simulink library "lib_AC_MSG"  (R2026a)
settings: Solver=VariableStepAuto
undefined symbols (not defined in the file): block_buses, block_idx, buses_lf, fref, Lbiginv, MSGs_buses, Nbuses, op_MSG, Ps_lf
settings Model: Creator=atomas  LastModifiedBy=atomas

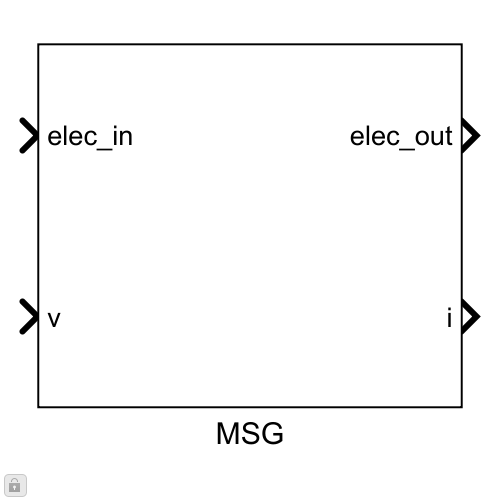
[thumbnail: Simulink's stored preview of the top-level diagram]
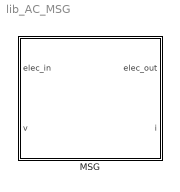
== system lib_AC_MSG ==
  MSG : Subsystem  mask(Doubly Fed Induction Generator){DFIGs_nodes=1, FBASE=50, D=0, H=7, Lssd_pu=1, Lssq_pu=0.6, Lmd_pu=0.9, Lmq_pu=0.5, Rs_pu=0.02, Lfd_pu=0.1, Rfd_pu=0.02, Rkd1_pu=10e6, Lkd1_pu=10e6, Rkd2_pu=10e6, Lkd2_pu=10e6, Rkq1_pu=10e6, Lkq1_pu=10e6, Rkq2_pu=10e6, Lkq2_pu=10e6, Rkq3_pu=10e6, Lkq3_pu=10e6, Ra_pu=0.008, La_pu=0.08, Cf_pu=0.0555, Ki_ia=0.1592, Kp_ia=9.1268e-04, Kid_m=1.9894, Kpd_m=0.0914, Kiq_m=1.1937, Kpq_m=0.0468, Ki_vc2=-0.1734, Kp_vc2=-0.0971, KPomegar=49, KIomegar=87.5, Kp_pll=9.1268e-05, Ki_pll=0.01592, T_e=1.15, T_1=12, T_2=1, T_A=0.01, K_A=200}
      mask prompts: FBASE "Base frequency (Hz)"; D "Damping (pu)"; H "Inertia (s)"; Lssd_pu "d-axis stator inductance (pu)"; Lssq_pu "q-axis stator inductance (pu)"; Lmd_pu "d-axis mutual inductance (pu)"; Lmq_pu "q-axis mutual inductance (pu)"; Rs_pu "Stator resistance (pu)"; Lfd_pu "Excitation indutance (pu)"; Rfd_pu "Excitation resistance (pu)"; Rkd1_pu "d-axis damper resistance 1 (pu)"; Lkd1_pu "d-axis damper inductance 1 (pu)"; Rkd2_pu "d-axis damper resistance 2 (pu)"; Lkd2_pu "d-axis damper inductance 2 (pu)"; Rkq1_pu "q-axis damper resistance 1(pu)"; Lkq1_pu "d-axis damper resistance 1 (pu)"; Rkq2_pu "d-axis damper resistance 2 (pu)"; Lkq2_pu "d-axis damper inductance 2 (pu)"; Rkq3_pu "d-axis damper resistance 3 (pu)"; Lkq3_pu "d-axis damper inductance 3 (pu)"; Ra_pu "Filter Resistance (pu)"; La_pu "Filter Inductance (pu)"; Cf_pu "DC-Link Capacitance"; Ki_ia "Grid side Converter Ki"; Kp_ia "Grid side Converter Kp"; Kid_m "d-axis Machine side Converter  Ki"; Kpd_m "d-axis Machine side Converter Kp"; Kiq_m "q-axis Machine side Converter  Ki"; Kpq_m "q-axis Machine side Converter Kp"; Ki_vc2 "DC Link Voltage Control Ki"; Kp_vc2 "DC Link Voltage Control Kp"; KPomegar "Speed control KP"; KIomegar "Speed control KI"; Kp_pll "PLL Kp"; Ki_pll "PLL Ki"
      mask help: Doubly Fed Induction Generator modelled in d-q reference frame.
      mask init:
      | [block_buses, block_idx, block_toM, block_fref, Lbiginv, Lssd_pu, Lssq_pu, Lmd_pu, Lfd_pu, La_pu, omega_base] = mask_init_MSG(gcb, FBASE, Lssd_pu, Lssq_pu, Lmd_pu, Lfd_pu, La_pu);
      mask Help: web([extractBefore(get_param(bdroot, 'filename'),gcs) 'Documentation/SM.html'])
      mask DialogControl Params Prompt: Parameters
      mask DialogControl Container10 Prompt: PI Parameters
      mask DialogControl Params_copy Prompt: Parameters
      mask DialogControl ContainerAVR Prompt: AVR Parameters
      mask DialogControl Params_AVR Prompt: Parameters

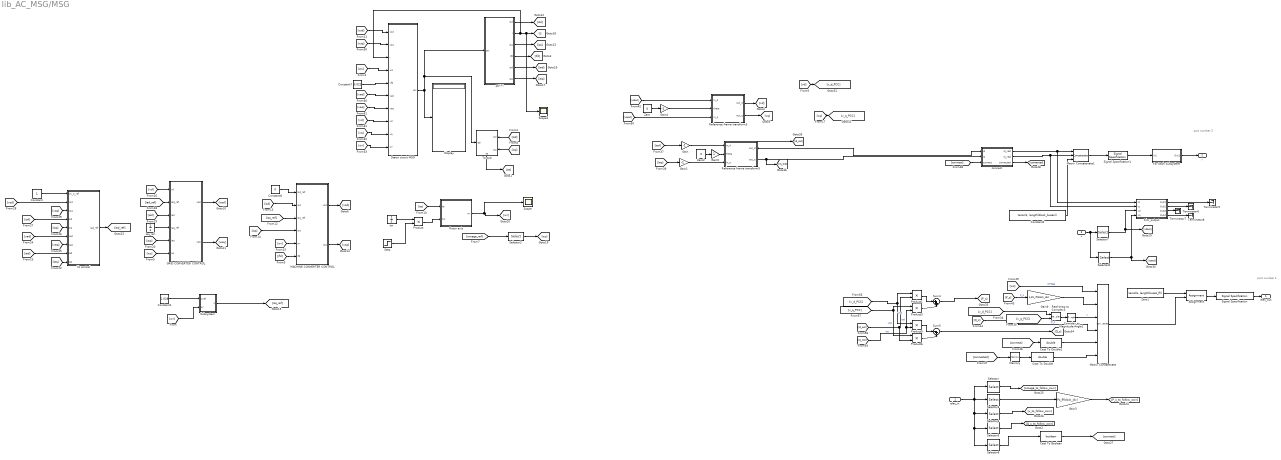
== system lib_AC_MSG/MSG ==
  note: port number 1
  note: port number 2
  elec_in : Inport
  v : Inport  Port=2
  Assignment : Assignment  NumberOfDimensions=2  DiagnosticForDimensions=Warning  IndexOptions=Assign all,Index vector (dialog)  Indices=1,block_idx  OutputSizes=1,1
  Cast To Boolean : DataTypeConversion  OutDataTypeStr=boolean  SaturateOnIntegerOverflow=off  RndMeth=Floor
  Cast To Double : DataTypeConversion  OutDataTypeStr=double  SaturateOnIntegerOverflow=off  RndMeth=Floor
  Cast To Double1 : DataTypeConversion  OutDataTypeStr=double  SaturateOnIntegerOverflow=off  RndMeth=Floor
  Complex to Magnitude-Angle1 : ComplexToMagnitudeAngle  Output=Magnitude
  Constant : Constant
  Constant1 : Constant  Value=1.028
  Constant2 : Constant  Value=zeros(1, length(block_buses))  VectorParams1D=off
  Constant6 : Constant  Value=0
  Constant7 : Constant  Value=0.022
  Display : Display
  For Each Subsystem : Subsystem  TreatAsAtomicUnit=on
  GRID CONVERTER CONTROL : Subsystem
  Gain : Gain  Gain=-1
  Gain1 : Gain  Gain=-1
  Gain3 : Gain  Gain=Ps_lf(block_idx)
  Gain4 : Gain  Gain=-1
  Gain5 : Gain
  Gain9 : Gain  Gain=1./Ps_lf(block_idx)
  MACHINE CONVERTER CONTROL : Subsystem
  Matrix Concatenate : Concatenate  NumInputs=6  Mode=Multidimensional array
  Matrix Concatenate1 : Concatenate  NumInputs=3  Mode=Multidimensional array
  Memory : Memory  InitialCondition=1
  Product{,1,3,5..6} (5 alike) : Product
  Real-Imag to Complex3 : RealImagToComplex
  Reference frame transform3 : Subsystem
  Reference frame transform5 : Subsystem
  Rotor axis : Subsystem
  Scope : Scope
      settings: ActiveDisplayYMinimum=1.0278  ActiveDisplayYMaximum=1.0294
  Scope1 : Scope
      settings: ActiveDisplayYMinimum=-1.2398  ActiveDisplayYMaximum=-0.95917  DataLoggingVariableName=ScopeData3
  Selector : Selector  NumberOfDimensions=2  InputPortWidth=3  IndexOptions=Index vector (dialog),Index vector (dialog)  Indices=1,block_idx  OutputSizes=1,1
  Selector2 : Selector  InputPortWidth=length(fref.ref_units)  IndexOptions=Index vector (dialog)  Indices=block_fref  OutputSizes=1
  Selector3 : Selector  NumberOfDimensions=2  InputPortWidth=3  IndexOptions=Index vector (dialog),Index vector (dialog)  Indices=2,block_idx  OutputSizes=1,1
  Selector4 : Selector  NumberOfDimensions=2  InputPortWidth=3  IndexOptions=Index vector (dialog),Index vector (dialog)  Indices=3,block_idx  OutputSizes=1,1
  Selector5 : Selector  NumberOfDimensions=2  InputPortWidth=3  IndexOptions=Index vector (dialog),Index vector (dialog)  Indices=4,block_idx  OutputSizes=1,1
  Selector6 : Selector  NumberOfDimensions=2  InputPortWidth=3  IndexOptions=Index vector (dialog),Index vector (dialog)  Indices=5,block_idx  OutputSizes=1,1
  Selector7 : Selector  NumberOfDimensions=2  InputPortWidth=3  IndexOptions=Index vector (dialog),Index vector (dialog)  Indices=1,block_buses  OutputSizes=1,1
  Selector8 : Selector  NumberOfDimensions=2  InputPortWidth=3  IndexOptions=Index vector (dialog),Index vector (dialog)  Indices=2,block_buses  OutputSizes=1,1
  Signal Specification : SignalSpecification  Dimensions=[6 length(buses_lf)]
  Signal Specification1 : SignalSpecification  Dimensions=[3 length(block_buses)]
  Stator circuit MSG : Subsystem
  Step : Step  InitialValue=1  FinalValue=1.1  SampleTime=0
  Subsystem : Subsystem
  Sum4 : Sum  Inputs=|++
  Sum5 : Sum  Inputs=|-+
  Terminator{5..8} (4 alike) : Terminator
  Torque : Subsystem
      settings: PortSchema="{\"entries\":[{\"content\":{\"sides\":[{\"content\":{\"connectorIds\":[\"In1\"]},\"type\":\"ConnectorPlacement.EquallySpacedRectSide\",\"uuid\":\"b7abd3bc-22dd-4669-aa40-98bc76884565\"},{\"content\":{\"connectorIds\":[\"In2\",\"In3\"],\"side\":\"RIGHT\"},\"type\":\"ConnectorPlacement.EquallySpacedRectSide\",\"uuid\":\"e9abb552-b46d-48ed-aa1f-0e9dac604fea\"},{\"content\":{\"connectorIds\":[],\"side\":\"TOP\"},\"type\":\"ConnectorPlacement.EquallySpacedRectSide\",\"uuid\":\"4b14997d-8f32-4cfb-8a1b-18cffb093d28\"},{\"content\":{\"connectorIds\":[\"Out1\"],\"side\":\"BOTTOM\"},\"type\":\"ConnectorPlacement.EquallySpacedRectSide\",\"uuid\":\"0ad577f8-eb9c-4d21-85f4-8d3c6640245c\"}]},\"type\":\"ConnectorPlacement.EquallySpacedConnector\",\"uuid\":\"d6624493-e930-4f0d-8cbe-17f96cb72edc\"}],\"packageUris\":[\"http://schema.mathworks.com/mf0/Connector/R2020b\"],\"version\":\"1.0\"}"
  Vc control : Subsystem
  Zero : Constant  Value=0  OutDataTypeStr=Inherit: Inherit via back propagation
  Zero1 : Constant  Value=zeros(6, length(buses_lf))  VectorParams1D=off  OutDataTypeStr=Inherit: Inherit via back propagation
  Zero2 : Constant  Value=0  OutDataTypeStr=Inherit: Inherit via back propagation
  connect : Subsystem
  iaq_ref : Integrator  InitialCondition=op_MSG.iaq_ref
  psi->i : Subsystem
  tm : Integrator  InitialCondition=op_MSG.tm
  trim_output : Subsystem
  elec_out : Outport
  i : Outport  Port=2
  wires:
  Product5/1 -> Sum5/1
  [v_d_PCC] -> Product1/1, Product5/1  "vod"
  Product3/1 -> Sum4/2
  [id_out] -> Product1/2, Product6/2  "iod"
  Sum5/1 -> [Q_s]
  [v_q_PCC] -> Product6/1, Product3/1  "voq"
  Product6/1 -> Sum5/2
  Sum4/1 -> [P_s]
  Product1/1 -> Sum4/1
  [iq_out] -> Product3/2, Product5/2  "ioq"
  Signal Specification/1 -> elec_out/1
  Gain4/1 -> Reference frame transform3/2(theta)
  For Each Subsystem/1(Out1) -> i/1
  [omega_ref] -> Selector2/1
  trim_output/2(Out2) -> Terminator6/1
  Selector5/1 -> [Q_s_to_follow_own]
  [iad] -> GRID CONVERTER CONTROL/3(iad)
  Vc control/1(iad_ref) -> [iad_ref]
  [vsd] -> Vc control/2(vsd)
  [vad] -> Vc control/6(vad)
  [te] -> Rotor axis/1(te)
  Assignment/1 -> Signal Specification/1
  GRID CONVERTER CONTROL/1(vad) -> [vad]
  [iaq] -> Vc control/9(iaq)
  GRID CONVERTER CONTROL/2(vaq) -> [vaq]
  [vsq] -> Vc control/3(vsq)
  psi->i/3(isq) -> [isq]
  [iad_ref] -> GRID CONVERTER CONTROL/2(iad_ref)
  Constant/1 -> Vc control/1(Vc_2_ref)
  iaq_ref/1 -> GRID CONVERTER CONTROL/4(iaq_ref)
  [iad] -> Vc control/8(iad)
  [vdout] -> Reference frame transform3/1(in_d)
  Zero/1 -> Gain4/1
  Gain9/1 -> Matrix Concatenate/2
  [P_s] -> Gain9/1  "P_s"
  Matrix Concatenate1/1 -> Signal Specification1/1
  trim_output/4(Out4) -> Terminator8/1
  Selector8/1 -> [vqout], trim_output/4(vq)
  Constant2/1 -> Matrix Concatenate1/3
  trim_output/3(Out3) -> Terminator7/1
  Cast To Boolean/1 -> [connect]
  v/1 -> Selector8/1, Selector7/1
  Signal Specification1/1 -> For Each Subsystem/1(In1)
  [vd] -> GRID CONVERTER CONTROL/1(vd)
  [ws] -> GRID CONVERTER CONTROL/6(ws)
  Selector7/1 -> trim_output/3(vd), [vdout]
  Gain5/1 -> Reference frame transform5/2(theta)
  elec_in/1 -> Selector6/1, Selector5/1, Selector4/1, Selector3/1, Selector/1
  connect/2(iq_real) -> trim_output/2(iq), Matrix Concatenate1/2
  [connect] -> Cast To Double1/1
  Cast To Double/1 -> Matrix Concatenate/6
  Cast To Double1/1 -> Matrix Concatenate/5
  Selector6/1 -> Cast To Boolean/1
  [Q_s] -> Matrix Concatenate/4  "Q_s"
  connect/1(id_real) -> trim_output/1(id), Matrix Concatenate1/1
  psi->i/2(i) -> Stator circuit MSG/3(i), Scope1/1, [i]
  trim_output/1(Out1) -> Terminator5/1
  [ws] -> Matrix Concatenate/1  "omega"
  Zero1/1 -> Assignment/1
  Selector/1 -> [omega_to_follow_own]
  Selector3/1 -> Gain3/1
  Selector4/1 -> [v_to_follow_own]
  Gain3/1 -> [P_s_to_follow_own]
  [vaq] -> Vc control/7(vaq)
  [isd] -> Vc control/4(isd)
  Matrix Concatenate/1 -> Assignment/2
  [iaq] -> GRID CONVERTER CONTROL/5(iaq)
  Zero2/1 -> Gain5/1
  psi->i/1(isd) -> [isd]
  [connect] -> connect/3(connect)
  [iad] -> Gain/1
  [connected] -> Memory/1
  [isq] -> Vc control/5(isq)
  connect/3(connected) -> [connected]
  Memory/1 -> Cast To Double/1
  Stator circuit MSG/1(psi) -> Torque/1(psi), psi->i/1(psi), Display/1
  Rotor axis/1(wr) -> Scope/1, [wr]
  Constant6/1 -> MACHINE CONVERTER CONTROL/1(isd_ref)
  [isq_ref] -> MACHINE CONVERTER CONTROL/3(isq_ref)
  MACHINE CONVERTER CONTROL/1(vsd) -> [vsd]
  [wr] -> MACHINE CONVERTER CONTROL/5(wr)
  MACHINE CONVERTER CONTROL/2(vsq) -> [vsq]
  Constant1/1 -> Subsystem/1(wref)
  [wr] -> Subsystem/2(wr)
  [ifd] -> MACHINE CONVERTER CONTROL/6(ifd)
  [vsd] -> Stator circuit MSG/1(vsd)
  [vsq] -> Stator circuit MSG/2(vsq)
  [vad] -> Stator circuit MSG/6(vad)
  [vaq] -> Stator circuit MSG/7(vaq)
  [ws] -> Stator circuit MSG/4(ws)
  [isd] -> Torque/2(isd)
  [isq] -> Torque/3(isq)
  Torque/1(te) -> [te]
  [vd] -> Stator circuit MSG/8(vd)
  [vq] -> Stator circuit MSG/9(vq)
  [wr] -> Stator circuit MSG/10(wr)
  [iaq] -> Gain1/1
  [v_q_PCC] -> Real-Imag to Complex3/2
  Real-Imag to Complex3/1 -> Complex to Magnitude-Angle1/1
  Complex to Magnitude-Angle1/1 -> Matrix Concatenate/3  "v"
  [v_d_PCC] -> Real-Imag to Complex3/1
  psi->i/5(iad) -> [iad]
  psi->i/6(iaq) -> [iaq]
  [vqout] -> Reference frame transform3/3(in_q)
  psi->i/4(ifd) -> [ifd]
  Constant7/1 -> Stator circuit MSG/5(vfd)
  Reference frame transform3/1(out_d) -> [vd]
  [vd] -> [v_d_PCC]
  Reference frame transform3/2(out_q) -> [vq]
  [vq] -> [v_q_PCC]
  Gain/1 -> Reference frame transform5/1(in_d)
  Gain1/1 -> Reference frame transform5/3(in_q)
  Reference frame transform5/1(out_d) -> [id_out], connect/1(id)
  Reference frame transform5/2(out_q) -> [iq_out], connect/2(iq)
  Subsystem/1(isq_ref) -> [isq_ref]
  [isd] -> MACHINE CONVERTER CONTROL/2(isd)
  [isq] -> MACHINE CONVERTER CONTROL/4(isq)
  tm/1 -> Product/1
  Step/1 -> Product/2
  Product/1 -> Rotor axis/2(tm)
  Selector2/1 -> [ws]

== system lib_AC_MSG/MSG/For Each Subsystem ==
  In1 : Inport  Partition=on  PartitionDimension=1  PartitionWidth=1  PartitionOffset=0
  Assignment : Assignment  DiagnosticForDimensions=Warning  IndexOptions=Index vector (dialog)  Indices=block_buses  OutputSizes=1
  For Each : ForEach  DisableCoverage=on
  Zero : Constant  Value=zeros(1,Nbuses)  VectorParams1D=off  OutDataTypeStr=Inherit: Inherit via back propagation
  Out1 : Outport  ConcatenationDimension=1
  wires:
  Assignment/1 -> Out1/1
  In1/1 -> Assignment/2
  Zero/1 -> Assignment/1

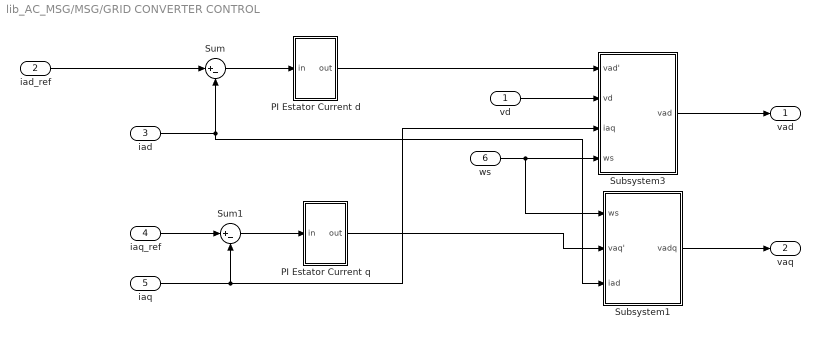
== system lib_AC_MSG/MSG/GRID CONVERTER CONTROL ==
  vd : Inport
  iad_ref : Inport  Port=2
  iad : Inport  Port=3
  iaq_ref : Inport  Port=4
  iaq : Inport  Port=5
  ws : Inport  Port=6
  PI Estator Current d : Subsystem
  PI Estator Current q : Subsystem
  Subsystem1 : Subsystem
  Subsystem3 : Subsystem
  Sum : Sum  Inputs=|+-
  Sum1 : Sum  Inputs=|+-
  vad : Outport  VectorParamsAs1DForOutWhenUnconnected=off
  vaq : Outport  Port=2  VectorParamsAs1DForOutWhenUnconnected=off
  wires:
  Subsystem1/1(vadq) -> vaq/1
  ws/1 -> Subsystem3/4(ws), Subsystem1/1(ws)
  iaq/1 -> Sum1/2, Subsystem3/3(iaq)
  iaq_ref/1 -> Sum1/1
  iad_ref/1 -> Sum/1
  Sum/1 -> PI Estator Current d/1(in)
  Sum1/1 -> PI Estator Current q/1(in)
  iad/1 -> Subsystem1/3(iad), Sum/2
  PI Estator Current d/1(out) -> Subsystem3/1(vad')
  PI Estator Current q/1(out) -> Subsystem1/2(vaq')
  vd/1 -> Subsystem3/2(vd)
  Subsystem3/1(vad) -> vad/1

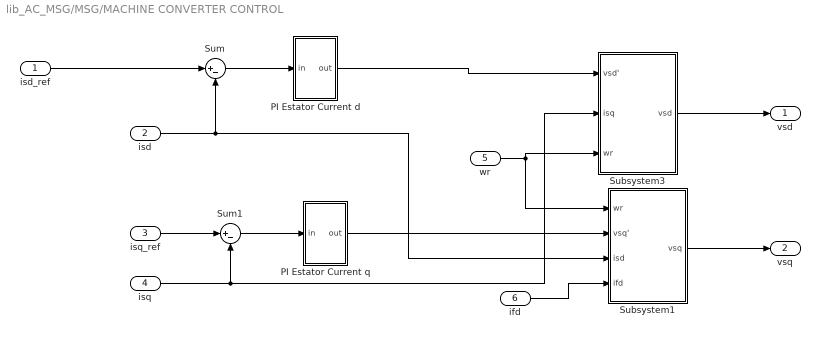
== system lib_AC_MSG/MSG/MACHINE CONVERTER CONTROL ==
  isd_ref : Inport
  isd : Inport  Port=2
  isq_ref : Inport  Port=3
  isq : Inport  Port=4
  wr : Inport  Port=5
  ifd : Inport  Port=6
  PI Estator Current d : Subsystem
  PI Estator Current q : Subsystem
  Subsystem1 : Subsystem
  Subsystem3 : Subsystem
  Sum : Sum  Inputs=|+-
  Sum1 : Sum  Inputs=|+-
  vsd : Outport  VectorParamsAs1DForOutWhenUnconnected=off
  vsq : Outport  Port=2  VectorParamsAs1DForOutWhenUnconnected=off
  wires:
  wr/1 -> Subsystem3/3(wr), Subsystem1/1(wr)
  isq/1 -> Sum1/2, Subsystem3/2(isq)
  isq_ref/1 -> Sum1/1
  isd_ref/1 -> Sum/1
  Sum/1 -> PI Estator Current d/1(in)
  Sum1/1 -> PI Estator Current q/1(in)
  isd/1 -> Subsystem1/3(isd), Sum/2
  PI Estator Current q/1(out) -> Subsystem1/2(vsq')
  Subsystem3/1(vsd) -> vsd/1
  ifd/1 -> Subsystem1/4(ifd)
  PI Estator Current d/1(out) -> Subsystem3/1(vsd')
  Subsystem1/1(vsq) -> vsq/1

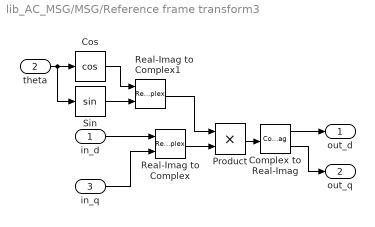
== system lib_AC_MSG/MSG/Reference frame transform3 ==
  in_d : Inport
  theta : Inport  Port=2
  in_q : Inport  Port=3
  Complex to Real-Imag : ComplexToRealImag
  Cos : Trigonometry  SCDEnableBlockLinearizationSpecification=on  Operator=cos
  Product : Product
  Real-Imag to Complex : RealImagToComplex
  Real-Imag to Complex1 : RealImagToComplex
  Sin : Trigonometry  SCDEnableBlockLinearizationSpecification=on
  out_d : Outport
  out_q : Outport  Port=2
  wires:
  Complex to Real-Imag/2 -> out_q/1
  Real-Imag to Complex1/1 -> Product/1
  Real-Imag to Complex/1 -> Product/2
  Product/1 -> Complex to Real-Imag/1
  theta/1 -> Sin/1, Cos/1
  Cos/1 -> Real-Imag to Complex1/1
  Sin/1 -> Real-Imag to Complex1/2
  Complex to Real-Imag/1 -> out_d/1
  in_q/1 -> Real-Imag to Complex/2
  in_d/1 -> Real-Imag to Complex/1

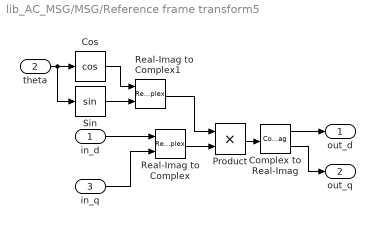
== system lib_AC_MSG/MSG/Reference frame transform5 ==
  in_d : Inport
  theta : Inport  Port=2
  in_q : Inport  Port=3
  Complex to Real-Imag : ComplexToRealImag
  Cos : Trigonometry  SCDEnableBlockLinearizationSpecification=on  Operator=cos
  Product : Product
  Real-Imag to Complex : RealImagToComplex
  Real-Imag to Complex1 : RealImagToComplex
  Sin : Trigonometry  SCDEnableBlockLinearizationSpecification=on
  out_d : Outport
  out_q : Outport  Port=2
  wires:
  in_d/1 -> Real-Imag to Complex/1
  in_q/1 -> Real-Imag to Complex/2
  Complex to Real-Imag/1 -> out_d/1
  Sin/1 -> Real-Imag to Complex1/2
  Cos/1 -> Real-Imag to Complex1/1
  theta/1 -> Cos/1, Sin/1
  Product/1 -> Complex to Real-Imag/1
  Real-Imag to Complex/1 -> Product/2
  Real-Imag to Complex1/1 -> Product/1
  Complex to Real-Imag/2 -> out_q/1

== system lib_AC_MSG/MSG/Rotor axis ==
  te : Inport
  tm : Inport  Port=2
  Gain : Gain  Gain=1/2./H
  Gain1 : Gain  Gain=D
  Sum1 : Sum  Inputs=-|+|-  InputSameDT=on  SaturateOnIntegerOverflow=on  OutDataTypeStr=Inherit: Same as first input
  \omega_r : Integrator  InitialCondition=op_MSG.Rotor_axis_omega_r  UpperSaturationLimit=2*pi  LowerSaturationLimit=0
  wr : Outport  VectorParamsAs1DForOutWhenUnconnected=off
  wires:
  Gain1/1 -> Sum1/3
  Gain/1 -> \omega_r/1
  Sum1/1 -> Gain/1
  te/1 -> Sum1/2
  \omega_r/1 -> Gain1/1, wr/1
  tm/1 -> Sum1/1

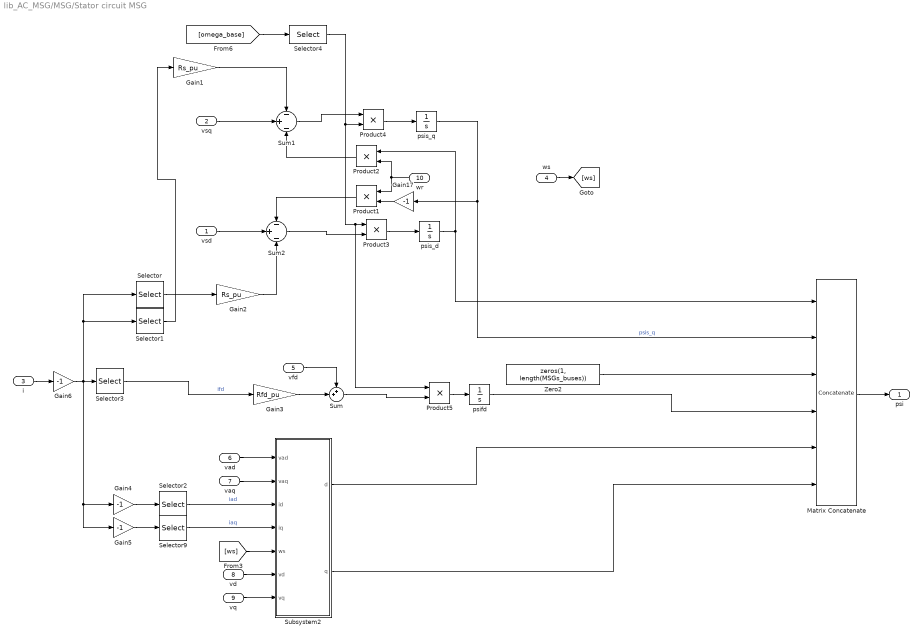
== system lib_AC_MSG/MSG/Stator circuit MSG ==
  vsd : Inport
  vsq : Inport  Port=2
  i : Inport  Port=3
  ws : Inport  Port=4
  vfd : Inport  Port=5
  vad : Inport  Port=6
  vaq : Inport  Port=7
  vd : Inport  Port=8
  vq : Inport  Port=9
  wr : Inport  Port=10
  Gain1 : Gain  Gain=Rs_pu
  Gain{4..6,17} (4 alike) : Gain  Gain=-1
  Gain2 : Gain  Gain=Rs_pu
  Gain3 : Gain  Gain=Rfd_pu
  Matrix Concatenate : Concatenate  NumInputs=6  Mode=Multidimensional array
  Product{1..5} (5 alike) : Product
  Selector : Selector  NumberOfDimensions=2  InputPortWidth=9  IndexOptions=Index vector (dialog),Select all  Indices=[1],1  OutputSizes=1,1
  Selector1 : Selector  NumberOfDimensions=2  InputPortWidth=9  IndexOptions=Index vector (dialog),Select all  Indices=[2],1  OutputSizes=1,1
  Selector2 : Selector  NumberOfDimensions=2  InputPortWidth=9  IndexOptions=Index vector (dialog),Select all  Indices=5,1  OutputSizes=1,1
  Selector3 : Selector  NumberOfDimensions=2  InputPortWidth=9  IndexOptions=Index vector (dialog),Select all  Indices=[4],1  OutputSizes=1,1
  Selector4 : Selector  InputPortWidth=length(fref.ref_units)  IndexOptions=Index vector (dialog)  Indices=block_fref  OutputSizes=1
  Selector9 : Selector  NumberOfDimensions=2  InputPortWidth=9  IndexOptions=Index vector (dialog),Select all  Indices=6,1  OutputSizes=1,1
  Subsystem2 : Subsystem
  Sum : Sum  Inputs=++|
  Sum1 : Sum  Inputs=-|+|-  InputSameDT=on  SaturateOnIntegerOverflow=on  OutDataTypeStr=Inherit: Same as first input
  Sum2 : Sum  Inputs=-|+|-  InputSameDT=on  SaturateOnIntegerOverflow=on  OutDataTypeStr=Inherit: Same as first input
  Zero2 : Constant  Value=zeros(1, length(MSGs_buses))  VectorParams1D=off  OutDataTypeStr=Inherit: Inherit via back propagation
  psifd : Integrator  InitialCondition=op_MSG.Stator_circuit_MSG_psifd
  psis_d : Integrator  InitialCondition=op_MSG.Stator_circuit_MSG_psis_d
  psis_q : Integrator  InitialCondition=op_MSG.Stator_circuit_MSG_psis_q
  psi : Outport  VectorParamsAs1DForOutWhenUnconnected=off
  wires:
  Product4/1 -> psis_q/1
  Sum1/1 -> Product4/1
  Gain3/1 -> Sum/2
  vfd/1 -> Sum/1
  Sum/1 -> Product5/2
  psifd/1 -> Matrix Concatenate/4
  Matrix Concatenate/1 -> psi/1
  Product5/1 -> psifd/1
  Zero2/1 -> Matrix Concatenate/3
  vsd/1 -> Sum2/2
  Sum2/1 -> Product3/2
  Product3/1 -> psis_d/1
  Gain17/1 -> Product1/2
  psis_q/1 -> Matrix Concatenate/2, Gain17/1  "psis_q"
  Product1/1 -> Sum2/1
  Product2/1 -> Sum1/3
  psis_d/1 -> Product2/1, Matrix Concatenate/1
  Gain2/1 -> Sum2/3
  Gain1/1 -> Sum1/1
  vsq/1 -> Sum1/2
  Selector9/1 -> Subsystem2/4(iq)  "iaq"
  Selector2/1 -> Subsystem2/3(id)  "iad"
  vad/1 -> Subsystem2/1(vad)
  Subsystem2/1(d) -> Matrix Concatenate/5
  Subsystem2/2(q) -> Matrix Concatenate/6
  vaq/1 -> Subsystem2/2(vaq)
  [ws] -> Subsystem2/5(ws)
  wr/1 -> Product1/1, Product2/2
  vq/1 -> Subsystem2/7(vq)
  vd/1 -> Subsystem2/6(vd)
  ws/1 -> [ws]
  i/1 -> Gain6/1
  Selector/1 -> Gain2/1
  Selector1/1 -> Gain1/1
  Gain4/1 -> Selector2/1
  Gain5/1 -> Selector9/1
  Selector3/1 -> Gain3/1  "ifd"
  Gain6/1 -> Gain5/1, Gain4/1, Selector/1, Selector1/1, Selector3/1
  Selector4/1 -> Product4/2, Product5/1, Product3/1
  [omega_base] -> Selector4/1

== system lib_AC_MSG/MSG/Subsystem ==
  wref : Inport
  wr : Inport  Port=2
  PI omega : Subsystem
  Sum : Sum  Inputs=|+-
  isq_ref : Outport
  wires:
  PI omega/1(out) -> isq_ref/1
  Sum/1 -> PI omega/1(in)
  wref/1 -> Sum/1
  wr/1 -> Sum/2

== system lib_AC_MSG/MSG/Torque ==
  psi : Inport
  isd : Inport  Port=2
  isq : Inport  Port=3
  Product1 : Product
  Product2 : Product
  Selector : Selector  NumberOfDimensions=2  InputPortWidth=9  IndexOptions=Index vector (dialog),Select all  Indices=[1],1  OutputSizes=1,1
  Selector1 : Selector  NumberOfDimensions=2  InputPortWidth=9  IndexOptions=Index vector (dialog),Select all  Indices=[2],1  OutputSizes=1,1
  Sum : Sum  Inputs=+||-
  te : Outport  VectorParamsAs1DForOutWhenUnconnected=off
  wires:
  Product1/1 -> Sum/1
  Sum/1 -> te/1
  Selector/1 -> Product1/1  "psistatordq"
  psi/1 -> Selector1/1, Selector/1
  Product2/1 -> Sum/2
  isq/1 -> Product1/2
  isd/1 -> Product2/1
  Selector1/1 -> Product2/2  "psistatordq"

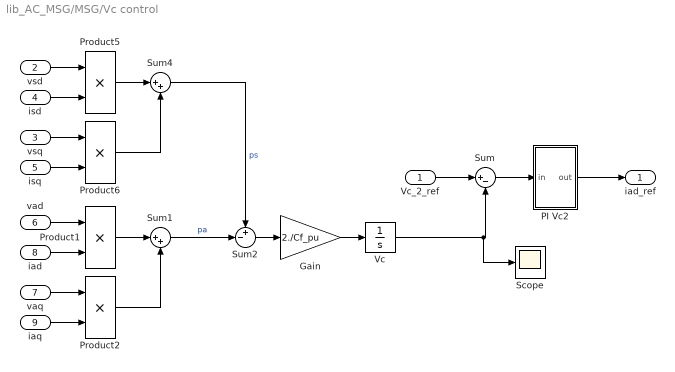
== system lib_AC_MSG/MSG/Vc control ==
  Vc_2_ref : Inport
  vsd : Inport  Port=2
  vsq : Inport  Port=3
  isd : Inport  Port=4
  isq : Inport  Port=5
  vad : Inport  Port=6
  vaq : Inport  Port=7
  iad : Inport  Port=8
  iaq : Inport  Port=9
  Gain : Gain  Gain=2./Cf_pu
  PI Vc2 : Subsystem
  Product{1..2,5..6} (4 alike) : Product
  Scope : Scope
      settings: ActiveDisplayYMinimum=0.13056  ActiveDisplayYMaximum=1.2418  DataLoggingVariableName=ScopeData2
  Sum : Sum  Inputs=|+-
  Sum1 : Sum  Inputs=|++
  Sum2 : Sum  Inputs=+-|
  Sum4 : Sum  Inputs=|++
  Vc : Integrator  InitialCondition=op_MSG.Vc_control_Vc
  iad_ref : Outport  VectorParamsAs1DForOutWhenUnconnected=off
  wires:
  Sum1/1 -> Sum2/2  "pa"
  Product1/1 -> Sum1/1
  Product2/1 -> Sum1/2
  vad/1 -> Product1/1
  vaq/1 -> Product2/1
  iaq/1 -> Product2/2
  iad/1 -> Product1/2
  Sum4/1 -> Sum2/1  "ps"
  isd/1 -> Product5/2
  isq/1 -> Product6/2
  vsq/1 -> Product6/1
  vsd/1 -> Product5/1
  Product6/1 -> Sum4/2
  Product5/1 -> Sum4/1
  Sum/1 -> PI Vc2/1(in)
  PI Vc2/1(out) -> iad_ref/1
  Sum2/1 -> Gain/1
  Vc/1 -> Scope/1, Sum/2
  Gain/1 -> Vc/1
  Vc_2_ref/1 -> Sum/1

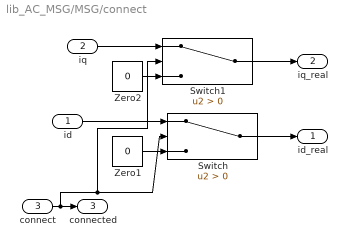
== system lib_AC_MSG/MSG/connect ==
  id : Inport
  iq : Inport  Port=2
  connect : Inport  Port=3
  Switch : Switch  Criteria=u2 > Threshold  ZeroCross=off  SaturateOnIntegerOverflow=off  InputSameDT=off
  Switch1 : Switch  Criteria=u2 > Threshold  ZeroCross=off  SaturateOnIntegerOverflow=off  InputSameDT=off
  Zero1 : Constant  Value=0  VectorParams1D=off  OutDataTypeStr=Inherit: Inherit via back propagation
  Zero2 : Constant  Value=0  VectorParams1D=off  OutDataTypeStr=Inherit: Inherit via back propagation
  id_real : Outport
  iq_real : Outport  Port=2
  connected : Outport  Port=3  OutDataTypeStr=boolean
  wires:
  Switch/1 -> id_real/1
  Zero1/1 -> Switch/3
  id/1 -> Switch/1
  connect/1 -> connected/1, Switch1/2, Switch/2
  Switch1/1 -> iq_real/1
  iq/1 -> Switch1/1
  Zero2/1 -> Switch1/3

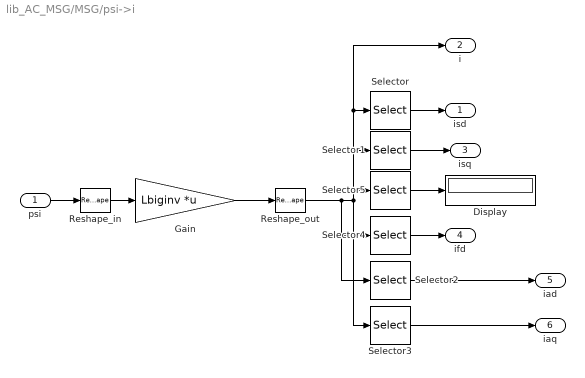
== system lib_AC_MSG/MSG/psi->i ==
  psi : Inport
  Display : Display
  Gain : Gain  Gain=Lbiginv  Multiplication=Matrix(K*u)
  Reshape_in : Reshape  OutputDimensionality=Column vector (2-D)
  Reshape_out : Reshape  OutputDimensionality=Customize  OutputDimensions=[6, length(MSGs_buses)]
  Selector : Selector  NumberOfDimensions=2  InputPortWidth=9  IndexOptions=Index vector (dialog),Select all  Indices=[1],1  OutputSizes=1,1
  Selector1 : Selector  NumberOfDimensions=2  InputPortWidth=9  IndexOptions=Index vector (dialog),Select all  Indices=[2],1  OutputSizes=1,1
  Selector2 : Selector  NumberOfDimensions=2  InputPortWidth=9  IndexOptions=Index vector (dialog),Select all  Indices=5,1  OutputSizes=1,1
  Selector3 : Selector  NumberOfDimensions=2  InputPortWidth=9  IndexOptions=Index vector (dialog),Select all  Indices=6,1  OutputSizes=1,1
  Selector4 : Selector  NumberOfDimensions=2  InputPortWidth=9  IndexOptions=Index vector (dialog),Select all  Indices=4,1  OutputSizes=1,1
  Selector5 : Selector  NumberOfDimensions=2  InputPortWidth=9  IndexOptions=Index vector (dialog),Select all  Indices=3,1  OutputSizes=1,1
  isd : Outport  VectorParamsAs1DForOutWhenUnconnected=off
  i : Outport  Port=2  VectorParamsAs1DForOutWhenUnconnected=off
  isq : Outport  Port=3  VectorParamsAs1DForOutWhenUnconnected=off
  ifd : Outport  Port=4  VectorParamsAs1DForOutWhenUnconnected=off
  iad : Outport  Port=5  VectorParamsAs1DForOutWhenUnconnected=off
  iaq : Outport  Port=6  VectorParamsAs1DForOutWhenUnconnected=off
  wires:
  Selector/1 -> isd/1
  Gain/1 -> Reshape_out/1
  psi/1 -> Reshape_in/1
  Reshape_in/1 -> Gain/1
  Selector1/1 -> isq/1
  Selector4/1 -> ifd/1
  Selector2/1 -> iad/1
  Selector3/1 -> iaq/1
  Reshape_out/1 -> Selector2/1, Selector4/1, i/1, Selector/1, Selector1/1, Selector5/1, Selector3/1
  Selector5/1 -> Display/1

== system lib_AC_MSG/MSG/trim_output ==
  id : Inport
  iq : Inport  Port=2
  vd : Inport  Port=3
  vq : Inport  Port=4
  Out1 : Outport
  Out2 : Outport  Port=2
  Out3 : Outport  Port=3
  Out4 : Outport  Port=4
  wires:
  id/1 -> Out1/1
  vq/1 -> Out4/1
  vd/1 -> Out3/1
  iq/1 -> Out2/1

== system lib_AC_MSG/MSG/GRID CONVERTER CONTROL/PI Estator Current d ==
  in : Inport
  Gain : Gain  Gain=Kp_ia
  Gain1 : Gain  Gain=Ki_ia
  Sum : Sum  Inputs=++|
  xa2 : Integrator  InitialCondition=op_MSG.GRID_CONVERTER_CONTROL_PI_Estator_Current_d_xa2
  out : Outport  VectorParamsAs1DForOutWhenUnconnected=off
  wires:
  xa2/1 -> Sum/2
  Gain/1 -> Sum/1
  in/1 -> Gain1/1, Gain/1
  Sum/1 -> out/1
  Gain1/1 -> xa2/1

== system lib_AC_MSG/MSG/GRID CONVERTER CONTROL/PI Estator Current q ==
  in : Inport
  Gain : Gain  Gain=Kp_ia
  Gain1 : Gain  Gain=Ki_ia
  Sum : Sum  Inputs=++|
  xa1 : Integrator  InitialCondition=op_MSG.GRID_CONVERTER_CONTROL_PI_Estator_Current_q_xa1
  out : Outport  VectorParamsAs1DForOutWhenUnconnected=off
  wires:
  Gain1/1 -> xa1/1
  Sum/1 -> out/1
  in/1 -> Gain/1, Gain1/1
  Gain/1 -> Sum/1
  xa1/1 -> Sum/2

== system lib_AC_MSG/MSG/GRID CONVERTER CONTROL/Subsystem1 ==
  ws : Inport
  vaq' : Inport  Port=2
  iad : Inport  Port=3
  Gain1 : Gain  Gain=La_pu
  Product1 : Product
  Sum4 : Sum  Inputs=-|-  InputSameDT=on  SaturateOnIntegerOverflow=on  OutDataTypeStr=Inherit: Same as first input
  vadq : Outport
  wires:
  iad/1 -> Product1/2
  Gain1/1 -> Product1/1
  vaq'/1 -> Sum4/1
  Sum4/1 -> vadq/1  "vadq"
  Product1/1 -> Sum4/2
  ws/1 -> Gain1/1

== system lib_AC_MSG/MSG/GRID CONVERTER CONTROL/Subsystem3 ==
  vad' : Inport
  vd : Inport  Port=2
  iaq : Inport  Port=3
  ws : Inport  Port=4
  Gain1 : Gain  Gain=La_pu
  Product1 : Product
  Sum4 : Sum  Inputs=-|+|+  InputSameDT=on  SaturateOnIntegerOverflow=on  OutDataTypeStr=Inherit: Same as first input
  vad : Outport
  wires:
  iaq/1 -> Product1/2
  ws/1 -> Gain1/1
  Product1/1 -> Sum4/3
  Sum4/1 -> vad/1  "vadq"
  vd/1 -> Sum4/2
  vad'/1 -> Sum4/1
  Gain1/1 -> Product1/1

== system lib_AC_MSG/MSG/MACHINE CONVERTER CONTROL/PI Estator Current d ==
  in : Inport
  Gain : Gain  Gain=Kpd_m
  Gain1 : Gain  Gain=Kid_m
  Sum : Sum  Inputs=++|
  xs1 : Integrator  InitialCondition=op_MSG.MACHINE_CONVERTER_CONTROL_PI_Estator_Current_d_xs1
  out : Outport  VectorParamsAs1DForOutWhenUnconnected=off
  wires:
  xs1/1 -> Sum/2
  Gain/1 -> Sum/1
  in/1 -> Gain1/1, Gain/1
  Sum/1 -> out/1
  Gain1/1 -> xs1/1

== system lib_AC_MSG/MSG/MACHINE CONVERTER CONTROL/PI Estator Current q ==
  in : Inport
  Gain : Gain  Gain=Kpq_m
  Gain1 : Gain  Gain=Kiq_m
  Sum : Sum  Inputs=++|
  xs2 : Integrator  InitialCondition=op_MSG.MACHINE_CONVERTER_CONTROL_PI_Estator_Current_q_xs2
  out : Outport  VectorParamsAs1DForOutWhenUnconnected=off
  wires:
  Gain1/1 -> xs2/1
  Sum/1 -> out/1
  in/1 -> Gain/1, Gain1/1
  Gain/1 -> Sum/1
  xs2/1 -> Sum/2

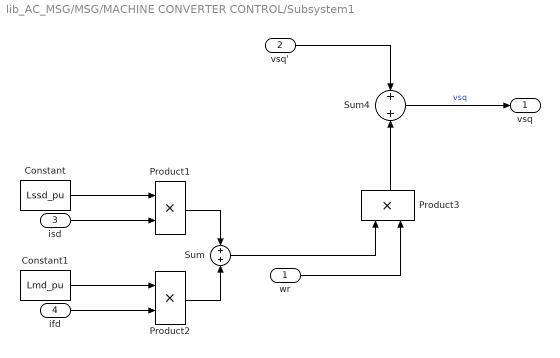
== system lib_AC_MSG/MSG/MACHINE CONVERTER CONTROL/Subsystem1 ==
  wr : Inport
  vsq' : Inport  Port=2
  isd : Inport  Port=3
  ifd : Inport  Port=4
  Constant : Constant  Value=Lssd_pu
  Constant1 : Constant  Value=Lmd_pu
  Product1 : Product
  Product2 : Product
  Product3 : Product
  Sum : Sum
  Sum4 : Sum  InputSameDT=on  SaturateOnIntegerOverflow=on  OutDataTypeStr=Inherit: Same as first input
  vsq : Outport
  wires:
  isd/1 -> Product1/2
  Constant/1 -> Product1/1
  vsq'/1 -> Sum4/1
  Sum4/1 -> vsq/1  "vsq"
  Constant1/1 -> Product2/1
  ifd/1 -> Product2/2
  Product1/1 -> Sum/1
  Product2/1 -> Sum/2
  wr/1 -> Product3/2
  Sum/1 -> Product3/1
  Product3/1 -> Sum4/2

== system lib_AC_MSG/MSG/MACHINE CONVERTER CONTROL/Subsystem3 ==
  vsd' : Inport
  isq : Inport  Port=2
  wr : Inport  Port=3
  Gain1 : Gain  Gain=Lssq_pu
  Product1 : Product
  Sum4 : Sum  Inputs=+|-  InputSameDT=on  SaturateOnIntegerOverflow=on  OutDataTypeStr=Inherit: Same as first input
  vsd : Outport
  wires:
  isq/1 -> Product1/2
  wr/1 -> Gain1/1
  Product1/1 -> Sum4/2
  Sum4/1 -> vsd/1  "vsd"
  vsd'/1 -> Sum4/1
  Gain1/1 -> Product1/1

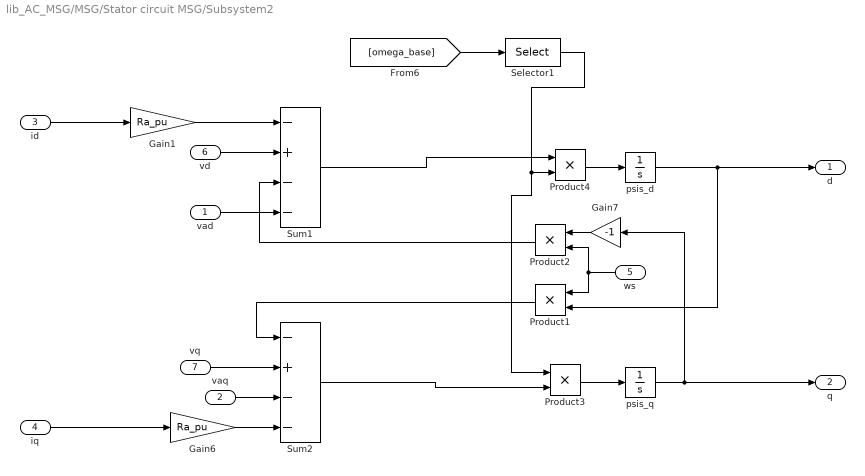
== system lib_AC_MSG/MSG/Stator circuit MSG/Subsystem2 ==
  vad : Inport
  vaq : Inport  Port=2
  id : Inport  Port=3
  iq : Inport  Port=4
  ws : Inport  Port=5
  vd : Inport  Port=6
  vq : Inport  Port=7
  Gain1 : Gain  Gain=Ra_pu
  Gain6 : Gain  Gain=Ra_pu
  Gain7 : Gain  Gain=-1
  Product{1..4} (4 alike) : Product
  Selector1 : Selector  InputPortWidth=length(fref.ref_units)  IndexOptions=Index vector (dialog)  Indices=block_fref  OutputSizes=1
  Sum1 : Sum  Inputs=-|+|-|-  InputSameDT=on  SaturateOnIntegerOverflow=on  OutDataTypeStr=Inherit: Same as first input
  Sum2 : Sum  Inputs=-|+|-|-  InputSameDT=on  SaturateOnIntegerOverflow=on  OutDataTypeStr=Inherit: Same as first input
  psis_d : Integrator  InitialCondition=op_MSG.Stator_circuit_MSG_Subsystem2_psis_d
  psis_q : Integrator  InitialCondition=op_MSG.Stator_circuit_MSG_Subsystem2_psis_q
  d : Outport
  q : Outport  Port=2
  wires:
  vaq/1 -> Sum2/3
  Product1/1 -> Sum2/1
  vq/1 -> Sum2/2
  Gain6/1 -> Sum2/4
  vad/1 -> Sum1/4
  vd/1 -> Sum1/2
  ws/1 -> Product1/1, Product2/2
  Product3/1 -> psis_q/1
  Product4/1 -> psis_d/1
  Gain1/1 -> Sum1/1
  psis_q/1 -> Gain7/1, q/1
  id/1 -> Gain1/1
  Product2/1 -> Sum1/3
  iq/1 -> Gain6/1
  Sum1/1 -> Product4/1
  Sum2/1 -> Product3/2
  psis_d/1 -> Product1/2, d/1
  Gain7/1 -> Product2/1
  Selector1/1 -> Product3/1, Product4/2
  [omega_base] -> Selector1/1

== system lib_AC_MSG/MSG/Subsystem/PI omega ==
  in : Inport
  Gain : Gain  Gain=KPomegar
  Gain1 : Gain  Gain=KIomegar
  Sum : Sum  Inputs=++|
  omegar : Integrator  InitialCondition=op_MSG.Subsystem_PI_omega_omegar
  out : Outport  VectorParamsAs1DForOutWhenUnconnected=off
  wires:
  omegar/1 -> Sum/2
  Gain/1 -> Sum/1
  in/1 -> Gain/1, Gain1/1
  Sum/1 -> out/1
  Gain1/1 -> omegar/1

== system lib_AC_MSG/MSG/Vc control/PI Vc2 ==
  in : Inport
  Gain : Gain  Gain=Kp_vc2
  Gain1 : Gain  Gain=Ki_vc2
  Sum : Sum  Inputs=++|
  xa3 : Integrator  InitialCondition=op_MSG.Vc_control_PI_Vc2_xa3
  out : Outport  VectorParamsAs1DForOutWhenUnconnected=off
  wires:
  Gain1/1 -> xa3/1
  Sum/1 -> out/1
  in/1 -> Gain/1, Gain1/1
  Gain/1 -> Sum/1
  xa3/1 -> Sum/2
